simulink model "InvertedP_test"  (R2025b)
settings: Solver=ode4  StartTime=0.0  StopTime=10.0  FixedStep=0.01  RelTol=1e-3
settings Model: Creator=MehrSystem  LastModifiedBy=MehrSystem

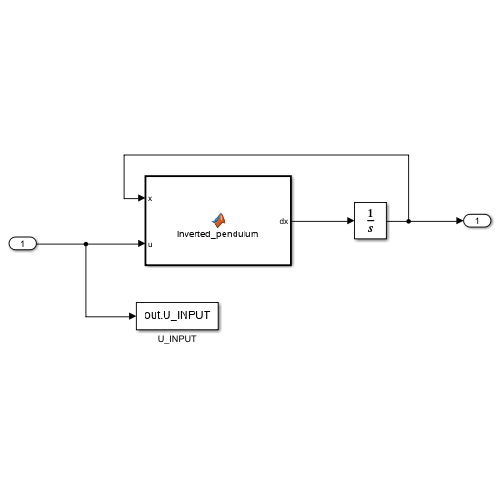
[thumbnail: Simulink's stored preview of the top-level diagram]
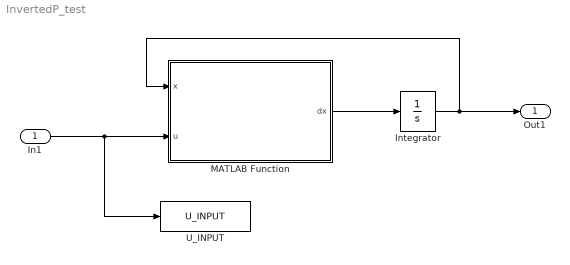
== system InvertedP_test ==
  In1 : Inport
  Integrator : Integrator  InitialCondition=[0 0]'
  MATLAB Function : MATLAB Function  TreatAsAtomicUnit=on
  U_INPUT : ToWorkspace  VariableName=U_INPUT  SaveFormat=Timeseries  SampleTime=-1
  Out1 : Outport
  wires:
  MATLAB Function/1(dx) -> Integrator/1
  Integrator/1 -> Out1/1, MATLAB Function/1(x)
  In1/1 -> U_INPUT/1, MATLAB Function/2(u)

== matlab function InvertedP_test/MATLAB Function ==
  data: x input; u input; dx output
function dx = inverted_pendulum(x, u)
    % Inverted pendulum continuous dynamics
    g = 9.81;
    l = 1.0;

    theta = x(1);
    theta_dot = x(2);

    theta_ddot = (g * sin(theta) - cos(theta) * u) / l;

    dx = [theta_dot; theta_ddot];
end
